simulink model "sf_bitwise_not_saturation"  (R2025b)
settings: Solver=FixedStepDiscrete  StartTime=0.0  StopTime=1  RelTol=1e-3  EnableMultiTasking=on
settings Model: Creator=The MathWorks, Inc.  LastModifiedBy=The MathWorks, Inc.
settings SolverCC: AlgebraicLoopSolver=TrustRegion
settings DataIOCC: ReturnWorkspaceOutputs=off
settings OptimizationCC: ReuseModelBlockBuffer=off  LifeSpan=inf
settings DebuggingCC: UnconnectedInputMsg=warning  UnconnectedOutputMsg=warning  UnconnectedLineMsg=warning  SymbolicDimsDataTypeCodeGenerationDiagnostic=none  SFUnexpectedBacktrackingDiag=warning  SFNoUnconditionalDefaultTransitionDiag=warning  ArithmeticOperatorsInVariantConditions=warning
settings ModelReferenceCC: EnableRefExpFcnMdlSchedulingChecks=on
settings SFSimCC: SimUseLocalCustomCode=off
settings RTWCC: RTWUseLocalCustomCode=off  GPUComputeCapability=3.5
settings CodeAppCC: StateflowObjectComments=on
settings GRTTargetCC: TargetLangStandard=C89/C90 (ANSI)
settings ConfigComp: CovMetricSettings=dw  CovSaveCumulativeToWorkspaceVar=on  CovSaveSingleToWorkspaceVar=on  CovExternalEMLEnable=off

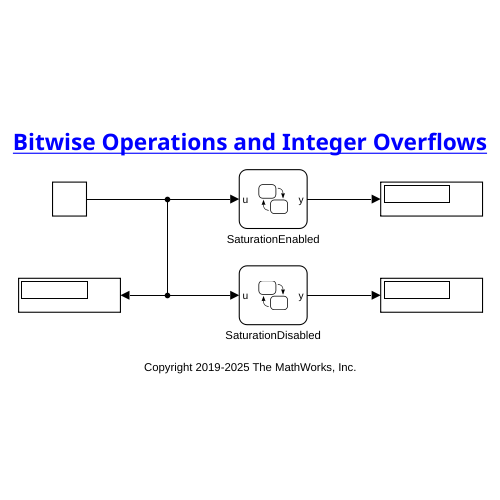
[thumbnail: Simulink's stored preview of the top-level diagram]
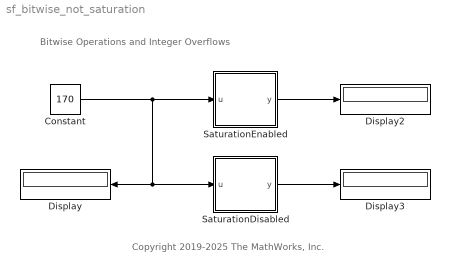
== system sf_bitwise_not_saturation ==
  note: Copyright 2019-2025 The MathWorks, Inc.
  note: Bitwise Operations and Integer Overflows
  Constant : Constant  Value=170  OutDataTypeStr=uint8
  Display : Display
      settings: Format=binary (Stored Integer)
  Display2 : Display
      settings: Format=binary (Stored Integer)
  Display3 : Display
      settings: Format=binary (Stored Integer)
  SaturationDisabled : Stateflow chart  TreatAsAtomicUnit=on
  SaturationEnabled : Stateflow chart  TreatAsAtomicUnit=on
  wires:
  Constant/1 -> Display/1, SaturationDisabled/1(u), SaturationEnabled/1(u)
  SaturationEnabled/1(y) -> Display2/1
  SaturationDisabled/1(y) -> Display3/1

== stateflow chart sf_bitwise_not_saturation/SaturationEnabled ==
  (default) -> (junction 2) : {y = ~u;}
  data: u input uint8 size=1; y output uint8 size=1

== stateflow chart sf_bitwise_not_saturation/SaturationDisabled ==
  (default) -> (junction 2) : {y = ~u;}
  data: u input uint8 size=1; y output uint8 size=1
